simulink model "exampleStateSpaceMult"  (R2019b)
settings: Solver=FixedStepAuto  StartTime=0.0  StopTime=100  FixedStep=0.008  RelTol=1e-3
values from neighbouring files (symbols this model uses):
  DT = 0.008    [LUTMFile.m]    (also in UIOLinestTr.m; exUIO_WECS.m; getFictInputMatricesOrd3M.m; initWorkspace.m)
  sysEst = c2d(ss(F,[T*B,K],eye(nx),[zeros(size(T*B)),H]),DT,'zoh')    [exUIO_WECS.m]
  sysEstCont = ss(F,[T*B,K],eye(nx),[zeros(size(T*B)),H])    [exUIO_WECS.m]
settings Model: Creator=ditt_aj  LastModifiedBy=ditt_aj

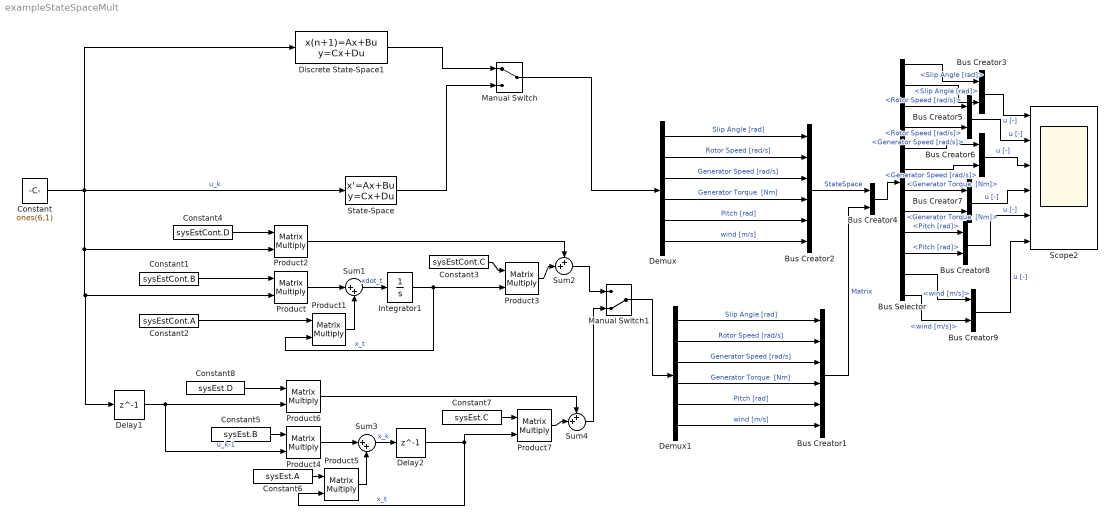
== system exampleStateSpaceMult ==
  Bus Creator1 : BusCreator  Inputs=6
  Bus Creator2 : BusCreator  Inputs=6
  Bus Creator{3..9} (7 alike) : BusCreator  Inputs=2
  Bus Selector : BusSelector  OutputSignals="StateSpace.Slip Angle [rad],Matrix.Slip Angle [rad],StateSpace.Rotor Speed [rad/s],Matrix.Rotor Speed [rad/s],StateSpace.Generator Speed [rad/s],Matrix.Generator Speed [rad/s],StateSpace.Generator Torque  [Nm],Matrix.Generator Torque  [Nm],StateSpace.Pitch [rad],Matrix.Pitch [rad],StateSpace.wind [m/s],Matrix.wind [m/s]"
  Constant : Constant  Value=ones(6,1)
  Constant1 : Constant  Value=sysEstCont.B
  Constant2 : Constant  Value=sysEstCont.A
  Constant3 : Constant  Value=sysEstCont.C
  Constant4 : Constant  Value=sysEstCont.D
  Constant5 : Constant  Value=sysEst.B
  Constant6 : Constant  Value=sysEst.A
  Constant7 : Constant  Value=sysEst.C
  Constant8 : Constant  Value=sysEst.D
  Delay1 : Delay  DelayLength=1
  Delay2 : Delay  DelayLength=1
  Demux : Demux  Outputs=6
  Demux1 : Demux  Outputs=6
  Discrete State-Space1 : DiscreteStateSpace  A=sysEst.A  B=sysEst.B  C=sysEst.C  D=sysEst.D  SampleTime=DT
  Integrator1 : Integrator
  Manual Switch : ManualSwitch
  Manual Switch1 : ManualSwitch  CurrentSetting=0
  Product{,1..7} (8 alike) : Product  Multiplication=Matrix(*)
  Scope2 : Scope  NumInputPorts=6
      settings: Tag=Scope
  State-Space : StateSpace  A=sysEstCont.A  B=sysEstCont.B  C=sysEstCont.C  D=sysEstCont.D  InitialCondition=0
  Sum1 : Sum  Inputs=|++
  Sum2 : Sum  Inputs=++|
  Sum3 : Sum  Inputs=|++
  Sum4 : Sum  Inputs=++|
  wires:
  Product/1 -> Sum1/1
  Product3/1 -> Sum2/2
  Product2/1 -> Sum2/1
  Sum1/1 -> Integrator1/1  "xdot_t"
  Integrator1/1 -> Product1/2, Product3/2  "x_t"
  Product1/1 -> Sum1/2
  Bus Creator2/1 -> Bus Creator4/1  "StateSpace"
  Bus Creator1/1 -> Bus Creator4/2  "Matrix"
  Constant1/1 -> Product/1
  Constant2/1 -> Product1/1
  Constant4/1 -> Product2/1
  Constant3/1 -> Product3/1
  Demux/1 -> Bus Creator2/1  "Slip Angle [rad]"
  Demux/6 -> Bus Creator2/6  "wind [m/s]"
  Demux/5 -> Bus Creator2/5  "Pitch [rad]"
  Demux/4 -> Bus Creator2/4  "Generator Torque  [Nm]"
  Demux/3 -> Bus Creator2/3  "Generator Speed [rad/s]"
  Demux/2 -> Bus Creator2/2  "Rotor Speed [rad/s]"
  Demux1/3 -> Bus Creator1/3  "Generator Speed [rad/s]"
  Demux1/5 -> Bus Creator1/5  "Pitch [rad]"
  Demux1/1 -> Bus Creator1/1  "Slip Angle [rad]"
  Demux1/2 -> Bus Creator1/2  "Rotor Speed [rad/s]"
  Demux1/4 -> Bus Creator1/4  "Generator Torque  [Nm]"
  Demux1/6 -> Bus Creator1/6  "wind [m/s]"
  Bus Creator4/1 -> Bus Selector/1
  Bus Selector/1 -> Bus Creator3/1  "<Slip Angle [rad]>"
  Bus Selector/2 -> Bus Creator3/2  "<Slip Angle [rad]>"
  Bus Creator3/1 -> Scope2/1  "u [-]"
  Bus Selector/3 -> Bus Creator5/1  "<Rotor Speed [rad/s]>"
  Bus Selector/4 -> Bus Creator5/2  "<Rotor Speed [rad/s]>"
  Bus Creator5/1 -> Scope2/2  "u [-]"
  Bus Selector/5 -> Bus Creator6/1  "<Generator Speed [rad/s]>"
  Bus Selector/6 -> Bus Creator6/2  "<Generator Speed [rad/s]>"
  Bus Creator6/1 -> Scope2/3  "u [-]"
  Bus Selector/7 -> Bus Creator7/1  "<Generator Torque  [Nm]>"
  Bus Selector/8 -> Bus Creator7/2  "<Generator Torque  [Nm]>"
  Bus Creator7/1 -> Scope2/4  "u [-]"
  Bus Selector/9 -> Bus Creator8/1  "<Pitch [rad]>"
  Bus Selector/10 -> Bus Creator8/2  "<Pitch [rad]>"
  Bus Creator8/1 -> Scope2/5  "u [-]"
  Bus Selector/11 -> Bus Creator9/1  "<wind [m/s]>"
  Bus Selector/12 -> Bus Creator9/2  "<wind [m/s]>"
  Bus Creator9/1 -> Scope2/6  "u [-]"
  Discrete State-Space1/1 -> Manual Switch/1
  State-Space/1 -> Manual Switch/2
  Manual Switch/1 -> Demux/1
  Product7/1 -> Sum4/2
  Delay2/1 -> Product5/2, Product7/2  "x_t"
  Sum3/1 -> Delay2/1  "x_k"
  Constant7/1 -> Product7/1
  Constant8/1 -> Product6/1
  Constant5/1 -> Product4/1
  Product6/1 -> Sum4/1
  Product4/1 -> Sum3/1
  Constant6/1 -> Product5/1
  Product5/1 -> Sum3/2
  Constant/1 -> Discrete State-Space1/1, State-Space/1, Product2/2, Delay1/1, Product/2  "u_k"
  Sum2/1 -> Manual Switch1/1
  Manual Switch1/1 -> Demux1/1
  Sum4/1 -> Manual Switch1/2
  Delay1/1 -> Product4/2, Product6/2  "u_k-1"
